simulink model "QD2_MissionCtrl_Dual_MPC"  (R2022b)
settings: Solver=ode2  StartTime=0.0  StopTime=inf  FixedStep=0.001  RelTol=1e-3  EnableMultiTasking=on
PreLoadFcn:
  | % Rutas: simulink_qdrone2 (qd2_cargar_config), lib (qd2_*.m) y la carpeta
  | % del modelo (QD2_Mission_Lib.slx de la misma versión de MATLAB).
  | qd2_d = fileparts(get_param(bdroot, 'FileName')); qd2_r = qd2_d;
  | while ~isempty(qd2_r) && ~exist(fullfile(qd2_r, 'qd2_cargar_config.m'), 'file')
  |     qd2_p = fileparts(qd2_r); if strcmp(qd2_p, qd2_r), qd2_r = ''; else, qd2_r = qd2_p; end
  | end
  | if ~isempty(qd2_r), addpath(fullfile(qd2_r, 'lib')); addpath(qd2_r); end
  | if exist(fullfile(qd2_d, 'QD2_Mission_Lib.slx'), 'file'), addpath(qd2_d); end
  | clear qd2_d qd2_r qd2_p
PostLoadFcn:
  | try, qd2_cargar_config(); catch qd2_e, warning(qd2_e.message); end
InitFcn:
  | qd2_cargar_config(bdroot);
undefined symbols (not defined in the file): _MissionCtrl, _MissionDual, datetime, Host, localhost, log_, m, qc_get_step_size, QD2CFG, QD2P, saved_data
libraries: quarc_library x43, QD2_Mission_Lib x12, simulink x11
(part 2 of 2)

== system QD2_MissionCtrl_Dual_MPC/MISSION CONTROL QDRONE POSITION CONTROL/Localization - Vicon ==
  note: Double-click on the Vicon block.
      |
      | Specify the Vicon Tracker server IP address and port number under Hostname field.
      |
      | Specify the object name corresponding to the vehicle to be tracked under the
      | List of segments field. The format for the segment is <ObjectName>.<ObjectName>
      | where <ObjectName> is the name given when defining the vehicle object in the
      | Vicon Tracker server softwre. Click the "+" button to add the name to the segment list
      | prior to clicking on the "OK" or "Apply" button.
      | Remove extra/unused entries from the list using the "-" button.
      |
      | Make sure the checkbox next to the Object name inside the Object tab in
      | Vicon Tracker software is selected/checked and Tracker is streaming (Live) tracking
      | data before running this model.
  Convention Correction (Vicon Frame to Research Studio Frame) : Subsystem  Commented=on
  For Each Subsystem (Convention Correction: Vicon Frame to Research Studio Frame) : Subsystem  TreatAsAtomicUnit=on
  Terminator{,1..4} (5 alike) : Terminator
  Vicon : quarc_library/Devices/Third-Party/Vicon/Vicon  hostname=localhost:801  segment_list=ObjectName1.ObjectName1\0\0  marker_list=\0  unlabeled_markers=[]  stream_mode=2  sample_time=qc_get_step_size  num_segments=1  num_markers=0  active=on
      settings: SourceProductName=QUARC Targets
  Data [7n] : Outport  VectorParamsAs1DForOutWhenUnconnected=off
  q [4n] : Outport  Port=2  VectorParamsAs1DForOutWhenUnconnected=off
  wires:
  Vicon/5 -> Terminator3/1
  Vicon/4 -> Terminator1/1
  Vicon/1 -> For Each Subsystem (Convention Correction: Vicon Frame to Research Studio Frame)/1(xyz_MF (m) [3n])
  Vicon/2 -> For Each Subsystem (Convention Correction: Vicon Frame to Research Studio Frame)/2(rot_MF (rad) [3n])
  Vicon/3 -> For Each Subsystem (Convention Correction: Vicon Frame to Research Studio Frame)/3(isTracking [n])
  For Each Subsystem (Convention Correction: Vicon Frame to Research Studio Frame)/5("data_RSF (m, rad, bool) [7n]") -> Data [7n]/1
  For Each Subsystem (Convention Correction: Vicon Frame to Research Studio Frame)/4(isTracking_RSF [n]) -> Terminator2/1
  For Each Subsystem (Convention Correction: Vicon Frame to Research Studio Frame)/3(rot_RSF (rad) [3n]) -> Terminator/1
  For Each Subsystem (Convention Correction: Vicon Frame to Research Studio Frame)/2(xyz_RSF (m) [3n]) -> Terminator4/1
  For Each Subsystem (Convention Correction: Vicon Frame to Research Studio Frame)/1(q_RSF [4n]) -> q [4n]/1

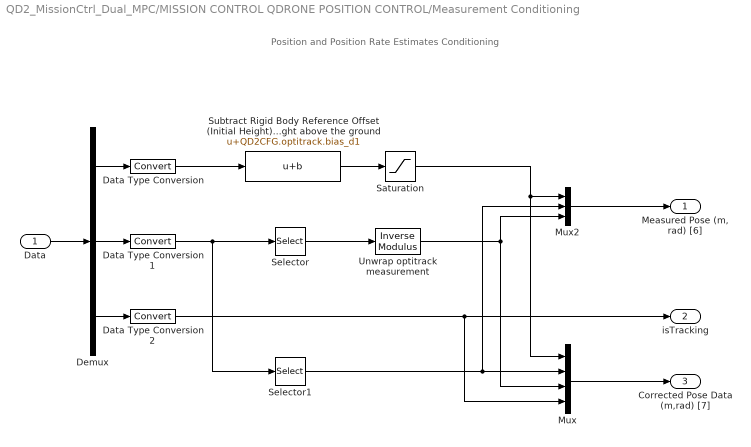
== system QD2_MissionCtrl_Dual_MPC/MISSION CONTROL QDRONE POSITION CONTROL/Measurement Conditioning ==
  note: Position and Position Rate Estimates Conditioning
  Data : Inport
  Data Type Conversion : DataTypeConversion  SaturateOnIntegerOverflow=off  RndMeth=Floor
  Data Type Conversion1 : DataTypeConversion  SaturateOnIntegerOverflow=off  RndMeth=Floor
  Data Type Conversion2 : DataTypeConversion  SaturateOnIntegerOverflow=off  RndMeth=Floor
  Demux : Demux  Outputs=[3 3 1]
  Mux : Mux
  Mux2 : Mux  Inputs=[3 2 1]
  Saturation : Saturate  UpperLimit=[2 2 5]  LowerLimit=[-2 -2 0]
  Selector : Selector  InputPortWidth=3  IndexOptions=Index vector (dialog)  Indices=[3]  OutputSizes=1
  Selector1 : Selector  InputPortWidth=3  IndexOptions=Index vector (dialog)  Indices=[1 2]  OutputSizes=1
  Subtract Rigid Body Reference Offset (Initial Height) to get height above the ground : Bias  Bias=QD2CFG.optitrack.bias_d1  SaturateOnIntegerOverflow=off
  Unwrap optitrack measurement : quarc_library/Discontinuities/Inverse Modulus  modulus=2*pi  output_derivative=off  output_revolutions=off  max_x=Inf  min_x=-Inf
  "Measured Pose (m, rad) [6]" : Outport  VectorParamsAs1DForOutWhenUnconnected=off
  isTracking : Outport  Port=2  VectorParamsAs1DForOutWhenUnconnected=off
  Corrected Pose Data (m,rad) [7] : Outport  Port=3  VectorParamsAs1DForOutWhenUnconnected=off
  wires:
  Demux/2 -> Data Type Conversion1/1
  Demux/1 -> Data Type Conversion/1
  Demux/3 -> Data Type Conversion2/1
  Mux2/1 -> "Measured Pose (m, rad) [6]"/1
  Data/1 -> Demux/1
  Data Type Conversion2/1 -> Mux/4, isTracking/1
  Subtract Rigid Body Reference Offset (Initial Height) to get height above the ground/1 -> Saturation/1
  Saturation/1 -> Mux2/1, Mux/1
  Data Type Conversion1/1 -> Selector1/1, Selector/1
  Selector/1 -> Unwrap optitrack measurement/1
  Data Type Conversion/1 -> Subtract Rigid Body Reference Offset (Initial Height) to get height above the ground/1
  Unwrap optitrack measurement/1 -> Mux2/3, Mux/3
  Mux/1 -> Corrected Pose Data (m,rad) [7]/1
  Selector1/1 -> Mux2/2, Mux/2

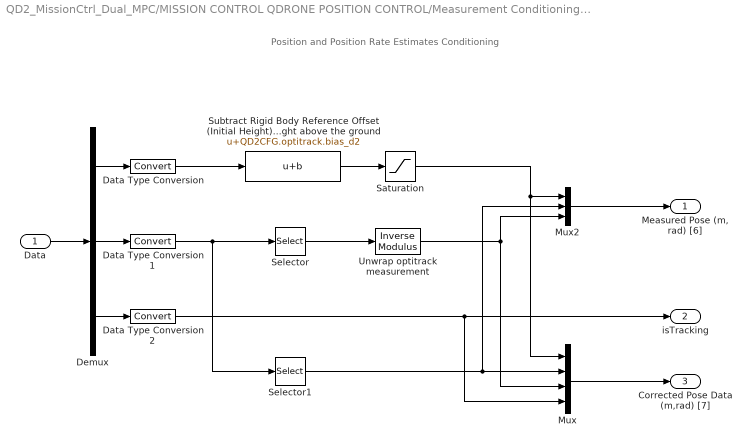
== system QD2_MissionCtrl_Dual_MPC/MISSION CONTROL QDRONE POSITION CONTROL/Measurement Conditioning QDrone 2 ==
  note: Position and Position Rate Estimates Conditioning
  Data : Inport
  Data Type Conversion : DataTypeConversion  SaturateOnIntegerOverflow=off  RndMeth=Floor
  Data Type Conversion1 : DataTypeConversion  SaturateOnIntegerOverflow=off  RndMeth=Floor
  Data Type Conversion2 : DataTypeConversion  SaturateOnIntegerOverflow=off  RndMeth=Floor
  Demux : Demux  Outputs=[3 3 1]
  Mux : Mux
  Mux2 : Mux  Inputs=[3 2 1]
  Saturation : Saturate  UpperLimit=[2 2 5]  LowerLimit=[-2 -2 0]
  Selector : Selector  InputPortWidth=3  IndexOptions=Index vector (dialog)  Indices=[3]  OutputSizes=1
  Selector1 : Selector  InputPortWidth=3  IndexOptions=Index vector (dialog)  Indices=[1 2]  OutputSizes=1
  Subtract Rigid Body Reference Offset (Initial Height) to get height above the ground : Bias  Bias=QD2CFG.optitrack.bias_d2  SaturateOnIntegerOverflow=off
  Unwrap optitrack measurement : quarc_library/Discontinuities/Inverse Modulus  modulus=2*pi  output_derivative=off  output_revolutions=off  max_x=Inf  min_x=-Inf
  "Measured Pose (m, rad) [6]" : Outport  VectorParamsAs1DForOutWhenUnconnected=off
  isTracking : Outport  Port=2  VectorParamsAs1DForOutWhenUnconnected=off
  Corrected Pose Data (m,rad) [7] : Outport  Port=3  VectorParamsAs1DForOutWhenUnconnected=off
  wires:
  Selector1/1 -> Mux/2, Mux2/2
  Mux/1 -> Corrected Pose Data (m,rad) [7]/1
  Unwrap optitrack measurement/1 -> Mux/3, Mux2/3
  Data Type Conversion/1 -> Subtract Rigid Body Reference Offset (Initial Height) to get height above the ground/1
  Selector/1 -> Unwrap optitrack measurement/1
  Data Type Conversion1/1 -> Selector/1, Selector1/1
  Saturation/1 -> Mux/1, Mux2/1
  Subtract Rigid Body Reference Offset (Initial Height) to get height above the ground/1 -> Saturation/1
  Data Type Conversion2/1 -> isTracking/1, Mux/4
  Data/1 -> Demux/1
  Mux2/1 -> "Measured Pose (m, rad) [6]"/1
  Demux/3 -> Data Type Conversion2/1
  Demux/1 -> Data Type Conversion/1
  Demux/2 -> Data Type Conversion1/1

== system QD2_MissionCtrl_Dual_MPC/MISSION CONTROL QDRONE POSITION CONTROL/Subsystem ==
  note: CORRECCIÓN (2 drones): el modelo de tierra ya no se detiene 3 s después de Land.
      | Stop Allowed (MISSION END CHECK) = los DOS drones en el suelo >= 3 s (o 60 s seguidos sin rastreo).
      | Después sigue el Delay original de 3 s y el Stop with Message.
  Joystick Signals (Boolean) : Inport
  "Communication Issue " : Inport  Port=2
  AND Stop Allowed : Logic  AllPortsSameDT=off  OutDataTypeStr=boolean
  Compare To Constant : simulink/Logic and Bit Operations/Compare To Constant  relop=>=  const=1  OutDataTypeStr=boolean
  Compare To Constant1 : simulink/Logic and Bit Operations/Compare To Constant  relop===  const=3  OutDataTypeStr=boolean
  Delay : Delay  DelayLength=3000
  Demux : Demux
  MATLAB Function : MATLAB Function  TreatAsAtomicUnit=on
  OR : Logic  Operator=OR  IconShape=distinctive  AllPortsSameDT=off  OutDataTypeStr=boolean
  Product : Product
  Stop with Message : quarc_library/Sinks/Error Handling/Stop with Message  message_type=Fixed error message  message_icon=Information  message=Mission plan ended, stopping mission control!
  Time : quarc_library/Sources/Time/Time  time_source=Wall clock  sample_time=qc_get_step_size
  Flight_State : Outport
  wires:
  Joystick Signals (Boolean)/1 -> Product/2
  Demux/1 -> MATLAB Function/1(Arm)
  Demux/2 -> MATLAB Function/2(Takeoff_Land_Flag)
  Demux/3 -> MATLAB Function/3(Emergency_Stop)
  Demux/4 -> MATLAB Function/4(Joystick_Issue)
  MATLAB Function/1(Flight_State) -> Flight_State/1, Compare To Constant1/1
  Product/1 -> Demux/1
  Time/1 -> Compare To Constant/1
  Compare To Constant/1 -> Product/1
  Delay/1 -> Stop with Message/1
  MATLAB Function/2(Stop_MS) -> OR/2
  Compare To Constant1/1 -> OR/1
  "Communication Issue "/1 -> MATLAB Function/5(Communication_Issue)
  OR/1 -> AND Stop Allowed/1
  [Stop_Allowed] -> AND Stop Allowed/2
  AND Stop Allowed/1 -> Delay/1

== system QD2_MissionCtrl_Dual_MPC/MISSION CONTROL QDRONE POSITION CONTROL/Subsystem QDrone 2 ==
  note: CORRECCIÓN (2 drones): el modelo de tierra ya no se detiene 3 s después de Land.
      | Stop Allowed (MISSION END CHECK) = los DOS drones en el suelo >= 3 s (o 60 s seguidos sin rastreo).
      | Después sigue el Delay original de 3 s y el Stop with Message.
  Joystick Signals (Boolean) : Inport
  "Communication Issue " : Inport  Port=2
  AND Stop Allowed : Logic  AllPortsSameDT=off  OutDataTypeStr=boolean
  Compare To Constant : simulink/Logic and Bit Operations/Compare To Constant  relop=>=  const=1  OutDataTypeStr=boolean
  Compare To Constant1 : simulink/Logic and Bit Operations/Compare To Constant  relop===  const=3  OutDataTypeStr=boolean
  Delay : Delay  DelayLength=3000
  Demux : Demux
  MATLAB Function : MATLAB Function  TreatAsAtomicUnit=on
  OR : Logic  Operator=OR  IconShape=distinctive  AllPortsSameDT=off  OutDataTypeStr=boolean
  Product : Product
  Stop with Message : quarc_library/Sinks/Error Handling/Stop with Message  message_type=Fixed error message  message_icon=Information  message=Mission plan ended, stopping mission control!
  Time : quarc_library/Sources/Time/Time  time_source=Wall clock  sample_time=qc_get_step_size
  Flight_State : Outport
  wires:
  AND Stop Allowed/1 -> Delay/1
  [Stop_Allowed] -> AND Stop Allowed/2
  OR/1 -> AND Stop Allowed/1
  "Communication Issue "/1 -> MATLAB Function/5(Communication_Issue)
  Compare To Constant1/1 -> OR/1
  MATLAB Function/2(Stop_MS) -> OR/2
  Delay/1 -> Stop with Message/1
  Compare To Constant/1 -> Product/1
  Time/1 -> Compare To Constant/1
  Product/1 -> Demux/1
  MATLAB Function/1(Flight_State) -> Compare To Constant1/1, Flight_State/1
  Demux/4 -> MATLAB Function/4(Joystick_Issue)
  Demux/3 -> MATLAB Function/3(Emergency_Stop)
  Demux/2 -> MATLAB Function/2(Takeoff_Land_Flag)
  Demux/1 -> MATLAB Function/1(Arm)
  Joystick Signals (Boolean)/1 -> Product/2

== system QD2_MissionCtrl_Dual_MPC/MISSION CONTROL QDRONE POSITION CONTROL/Triggered Subsystem ==
  note: This looks for the first falling edge of the communication issue before allowing a communication issue to be triggered,
      | because the mission server model starts first.
  Trigger : TriggerPort  TriggerType=falling  VariantControl=Variant
  Add : Sum
  Compare To Constant : simulink/Logic and Bit Operations/Compare To Constant  relop=>=  const=1  OutDataTypeStr=boolean
  Constant : Constant
  Memory : Memory  InheritSampleTime=on
  Communication Issue (0,1) : Outport  InitialOutput=0  VectorParamsAs1DForOutWhenUnconnected=off
  wires:
  Constant/1 -> Add/1
  Memory/1 -> Add/2
  Add/1 -> Compare To Constant/1, Memory/1
  Compare To Constant/1 -> Communication Issue (0,1)/1

== system QD2_MissionCtrl_Dual_MPC/MISSION CONTROL QDRONE POSITION CONTROL/Triggered Subsystem QDrone 2 ==
  note: This looks for the first falling edge of the communication issue before allowing a communication issue to be triggered,
      | because the mission server model starts first.
  Trigger : TriggerPort  TriggerType=falling  VariantControl=Variant
  Add : Sum
  Compare To Constant : simulink/Logic and Bit Operations/Compare To Constant  relop=>=  const=1  OutDataTypeStr=boolean
  Constant : Constant
  Memory : Memory  InheritSampleTime=on
  Communication Issue (0,1) : Outport  InitialOutput=0  VectorParamsAs1DForOutWhenUnconnected=off
  wires:
  Compare To Constant/1 -> Communication Issue (0,1)/1
  Add/1 -> Memory/1, Compare To Constant/1
  Memory/1 -> Add/2
  Constant/1 -> Add/1

== system QD2_MissionCtrl_Dual_MPC/MISSION CONTROL QDRONE POSITION CONTROL/Waypoint Trajectories ==
  note: Add waypoints as multiple rows of the RED matrix. The amount of time to wait at each waypoint is is defined as the coloumns of the GREEN row matrix.
      |
      | When Enable goes high, the vehicle will move to the first waypoint and wait there.
      | When Play/Pause goes high, the vehicle will spend time at the first waypoint (specified in the time vector) and then proceed to cycle through the remaining waypoints.
      | When Play/Pause goes low, the vehicle will pause at the current waypoint. If Play/Pause goes high again, it will resume by spending time at the corresponding waypoint
      | as specified in the time vector all over again.
      | When Enable goes low at any point, the vehicle will move back to the Default pose.
  Play/Pause : Inport
  "Default (m, rad) [4]" : Inport  Port=2
  Drone Pose (m,rad) [4] : Inport  Port=3
  Each row is a pose (Multiple rows are multiple poses) : Constant  Value=[0,0,1.0,0;-1.5,-1.5,1.0,0; 0,-1.5,1.0,0; 1.5,-1.5,1.0,0; -1.5,1.5,1.0,0;0 1.5 1.0 0; 1.5 1.5 1.0 0; 1.5 0.75 1.0 0; 0,0,1.0,0]  VectorParams1D=off
  Switch : Switch  Criteria=u2 > Threshold  SaturateOnIntegerOverflow=off  InputSameDT=off
  Waiting per location (s) (number of entries matches number of rows in position matrix above) : Constant  Value=5
  Waypoint_Generator : Subsystem
  Finished (0,1) : Outport
  "Trajectory (m, rad) [4]" : Outport  Port=2
  wires:
  Waypoint_Generator/2(Finished (0,1)) -> Finished (0,1)/1
  Switch/1 -> "Trajectory (m, rad) [4]"/1
  "Default (m, rad) [4]"/1 -> Switch/3
  Waypoint_Generator/1(Pose) -> Switch/1
  Play/Pause/1 -> Switch/2
  Each row is a pose (Multiple rows are multiple poses)/1 -> Waypoint_Generator/1(Pose Matrix)
  Drone Pose (m,rad) [4]/1 -> Waypoint_Generator/2(Drone Pose)
  Waiting per location (s) (number of entries matches number of rows in position matrix above)/1 -> Waypoint_Generator/3(Wait time)

== system QD2_MissionCtrl_Dual_MPC/MISSION CONTROL QDRONE POSITION CONTROL/Calculate Home Pose/Enabled Subsystem ==
  "Pose (m, rad ) [4] " : Inport
  Enable : EnablePort
  "Home Pose (m, rad ) [4]" : Outport  VectorParamsAs1DForOutWhenUnconnected=off
  wires:
  "Pose (m, rad ) [4] "/1 -> "Home Pose (m, rad ) [4]"/1

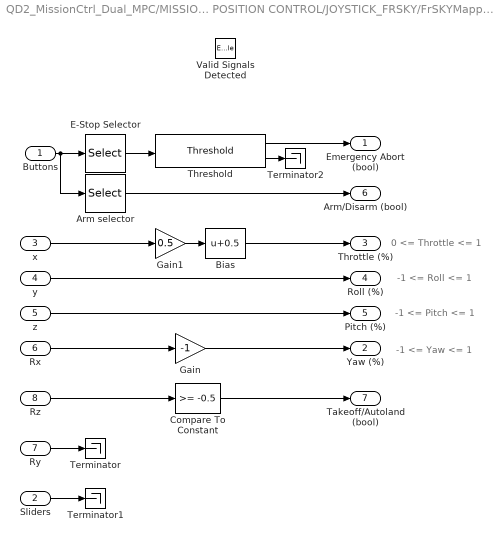
== system QD2_MissionCtrl_Dual_MPC/MISSION CONTROL QDRONE POSITION CONTROL/JOYSTICK_FRSKY/FrSKYMapping ==
  note: -1 <= Yaw <= 1
  note: 0 <= Throttle <= 1
  note: -1 <= Roll <= 1
  note: -1 <= Pitch <= 1
  Buttons : Inport
  Sliders : Inport  Port=2
  x : Inport  Port=3
  y : Inport  Port=4
  z : Inport  Port=5
  Rx : Inport  Port=6
  Ry : Inport  Port=7
  Rz : Inport  Port=8
  Valid Signals Detected : EnablePort
  Arm selector : Selector  InputPortWidth=32  IndexOptions=Index vector (dialog)  Indices=[2]  OutputSizes=1
  Bias : Bias  Bias=0.5  SaturateOnIntegerOverflow=off
  Compare To Constant : simulink/Logic and Bit Operations/Compare To Constant  relop=>=  const=-0.5  OutDataTypeStr=boolean
  E-Stop Selector : Selector  InputPortWidth=32  IndexOptions=Index vector (dialog)  Indices=[1]  OutputSizes=1
  Gain : Gain  Gain=-1
  Gain1 : Gain  Gain=0.5
  Terminator : Terminator
  Terminator1 : Terminator
  Terminator2 : Terminator
  Threshold : quarc_library/Discontinuities/Threshold  operator=>=  param_src=Specify via dialog  threshold=0.5  duration=0.2
      settings: SourceProductName=QUARC Targets
  Emergency Abort (bool) : Outport  VectorParamsAs1DForOutWhenUnconnected=off
  Yaw (%) : Outport  Port=2  VectorParamsAs1DForOutWhenUnconnected=off
  Throttle (%) : Outport  Port=3  VectorParamsAs1DForOutWhenUnconnected=off
  Roll (%) : Outport  Port=4  VectorParamsAs1DForOutWhenUnconnected=off
  Pitch (%) : Outport  Port=5  VectorParamsAs1DForOutWhenUnconnected=off
  "Arm/Disarm (bool) " : Outport  Port=6  VectorParamsAs1DForOutWhenUnconnected=off
  Takeoff/Autoland (bool) : Outport  Port=7  VectorParamsAs1DForOutWhenUnconnected=off
  wires:
  Buttons/1 -> Arm selector/1, E-Stop Selector/1
  Arm selector/1 -> "Arm/Disarm (bool) "/1
  x/1 -> Gain1/1
  y/1 -> Roll (%)/1
  z/1 -> Pitch (%)/1
  Rx/1 -> Gain/1
  Ry/1 -> Terminator/1
  Sliders/1 -> Terminator1/1
  E-Stop Selector/1 -> Threshold/1
  Rz/1 -> Compare To Constant/1
  Compare To Constant/1 -> Takeoff/Autoland (bool)/1
  Threshold/1 -> Emergency Abort (bool)/1
  Threshold/2 -> Terminator2/1
  Gain/1 -> Yaw (%)/1
  Gain1/1 -> Bias/1
  Bias/1 -> Throttle (%)/1

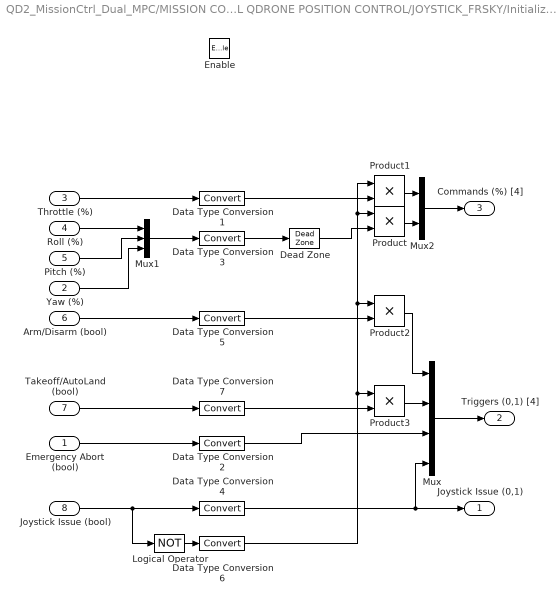
== system QD2_MissionCtrl_Dual_MPC/MISSION CONTROL QDRONE POSITION CONTROL/JOYSTICK_FRSKY/Initialization and Conditioning ==
  Emergency Abort (bool) : Inport
  Yaw (%) : Inport  Port=2
  Throttle (%) : Inport  Port=3
  Roll (%) : Inport  Port=4
  Pitch (%) : Inport  Port=5
  Arm/Disarm (bool) : Inport  Port=6
  Takeoff/AutoLand (bool) : Inport  Port=7
  Joystick Issue (bool) : Inport  Port=8
  Enable : EnablePort  StatesWhenEnabling=reset
  Data Type Conversion{1..7} (7 alike) : DataTypeConversion  SaturateOnIntegerOverflow=off  RndMeth=Floor
  Dead Zone : DeadZone  LowerValue=-0.01  UpperValue=0.01
  Logical Operator : Logic  Operator=NOT  AllPortsSameDT=off  OutDataTypeStr=boolean
  Mux : Mux
  Mux1 : Mux  Inputs=3
  Mux2 : Mux  Inputs=2
  Product{,1..3} (4 alike) : Product
  Joystick Issue (0,1) : Outport  InitialOutput=0  VectorParamsAs1DForOutWhenUnconnected=off
  Triggers (0,1) [4] : Outport  Port=2  InitialOutput=0  VectorParamsAs1DForOutWhenUnconnected=off
  Commands (%) [4] : Outport  Port=3  InitialOutput=0  VectorParamsAs1DForOutWhenUnconnected=off
  wires:
  Joystick Issue (bool)/1 -> Data Type Conversion4/1, Logical Operator/1
  Mux1/1 -> Data Type Conversion3/1
  Throttle (%)/1 -> Data Type Conversion1/1
  Roll (%)/1 -> Mux1/1
  Pitch (%)/1 -> Mux1/2
  Yaw (%)/1 -> Mux1/3
  Data Type Conversion4/1 -> Mux/4, Joystick Issue (0,1)/1
  Emergency Abort (bool)/1 -> Data Type Conversion2/1
  Data Type Conversion3/1 -> Dead Zone/1
  Arm/Disarm (bool)/1 -> Data Type Conversion5/1
  Mux/1 -> Triggers (0,1) [4]/1
  Data Type Conversion2/1 -> Mux/3
  Logical Operator/1 -> Data Type Conversion6/1
  Product/1 -> Mux2/2
  Product1/1 -> Mux2/1
  Data Type Conversion1/1 -> Product1/2
  Dead Zone/1 -> Product/2
  Data Type Conversion6/1 -> Product1/1, Product/1, Product2/1, Product3/1
  Product2/1 -> Mux/1
  Data Type Conversion5/1 -> Product2/2
  Takeoff/AutoLand (bool)/1 -> Data Type Conversion7/1
  Product3/1 -> Mux/2
  Data Type Conversion7/1 -> Product3/2
  Mux2/1 -> Commands (%) [4]/1

== system QD2_MissionCtrl_Dual_MPC/MISSION CONTROL QDRONE POSITION CONTROL/JOYSTICK_FRSKY/Pulse Check ==
  note: For this subsystem we will count the number of new pulses. The data can be considered enabled once the count of new signals has gone beyond 2. This will enable the Initializing and conditioning subsystem.
  new : Inport
  Compare : quarc_library/Logic Operations/Compare  operator=>=  output_data_type=boolean
      settings: SourceProductName=QUARC Targets
  Pulse Check : Constant
  "pulse count " : Subsystem  TreatAsAtomicUnit=on
  signal enable : Outport  InitialOutput=0  VectorParamsAs1DForOutWhenUnconnected=off
  wires:
  Compare/1 -> signal enable/1
  Pulse Check/1 -> Compare/2
  new/1 -> "pulse count "/Trigger
  "pulse count "/1(Number of Pulses) -> Compare/1

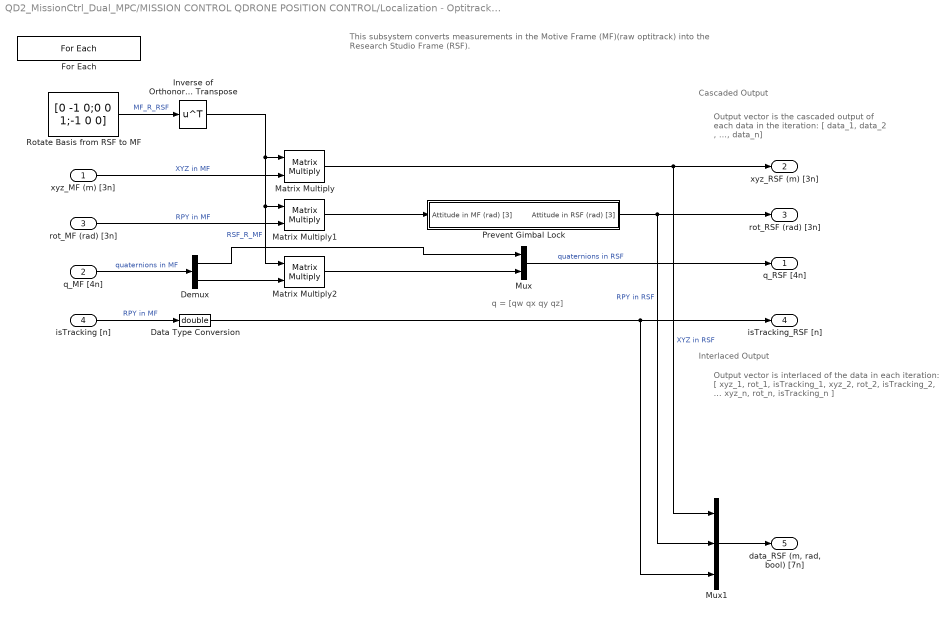
== system QD2_MissionCtrl_Dual_MPC/MISSION CONTROL QDRONE POSITION CONTROL/Localization - Optitrack/For Each Subsystem (Convention Correction: Motive Frame to Research Studio Frame) ==
  note: Output vector is interlaced of the data
      | in each iteration:
      |
      | [ xyz_1, rot_1, isTracking_1,
      |   xyz_2, rot_2, isTracking_2,
      |   ...
      |   xyz_n, rot_n, isTracking_n ]
  note: Interlaced Output
  note: Output vector is the cascaded output of
      | each data in the iteration:
      | [ data_1, data_2 , ..., data_n]
  note: Cascaded Output
  note: q = [qw qx qy qz]
  note: This subsystem converts measurements in the Motive Frame (MF)(raw optitrack) into the Research Studio Frame (RSF).
  xyz_MF (m) [3n] : Inport  Partition=on  PartitionDimension=1  PartitionWidth=3  PartitionOffset=0
  q_MF [4n] : Inport  Port=2  Partition=on  PartitionDimension=1  PartitionWidth=4  PartitionOffset=0
  rot_MF (rad) [3n] : Inport  Port=3  Partition=on  PartitionDimension=1  PartitionWidth=3  PartitionOffset=0
  isTracking [n] : Inport  Port=4  Partition=on  PartitionDimension=1  PartitionWidth=1  PartitionOffset=0
  Data Type Conversion : DataTypeConversion  OutDataTypeStr=double  SaturateOnIntegerOverflow=off  RndMeth=Floor
  Demux : Demux  Outputs=[1 3]
  For Each : ForEach  DisableCoverage=on
  Inverse of Orthonormal Matrix is its Transpose : Math  Operator=transpose
  Matrix Multiply : Product  Multiplication=Matrix(*)
  Matrix Multiply1 : Product  Multiplication=Matrix(*)
  Matrix Multiply2 : Product  Multiplication=Matrix(*)
  Mux : Mux  Inputs=2
  Mux1 : Mux  Inputs=3
  Prevent Gimbal Lock : Subsystem
  Rotate Basis from RSF to MF : Constant  Value=[0 -1 0;0 0 1;-1 0 0]
  q_RSF [4n] : Outport  ConcatenationDimension=1
  xyz_RSF (m) [3n] : Outport  Port=2  ConcatenationDimension=1
  rot_RSF (rad) [3n] : Outport  Port=3  ConcatenationDimension=1
  isTracking_RSF [n] : Outport  Port=4  ConcatenationDimension=1
  "data_RSF (m, rad, bool) [7n]" : Outport  Port=5  ConcatenationDimension=1
  wires:
  Mux/1 -> q_RSF [4n]/1  "quaternions in RSF"
  Demux/1 -> Mux/1
  Matrix Multiply2/1 -> Mux/2
  Demux/2 -> Matrix Multiply2/2
  q_MF [4n]/1 -> Demux/1  "quaternions in MF"
  Prevent Gimbal Lock/1(Attitude in RSF (rad) [3]) -> Mux1/2, rot_RSF (rad) [3n]/1  "RPY in RSF"
  Matrix Multiply1/1 -> Prevent Gimbal Lock/1(Attitude in MF (rad) [3])
  rot_MF (rad) [3n]/1 -> Matrix Multiply1/2  "RPY in MF"
  Matrix Multiply/1 -> Mux1/1, xyz_RSF (m) [3n]/1  "XYZ in RSF"
  Inverse of Orthonormal Matrix is its Transpose/1 -> Matrix Multiply/1, Matrix Multiply1/1, Matrix Multiply2/1  "RSF_R_MF"
  xyz_MF (m) [3n]/1 -> Matrix Multiply/2  "XYZ in MF"
  Rotate Basis from RSF to MF/1 -> Inverse of Orthonormal Matrix is its Transpose/1  "MF_R_RSF"
  isTracking [n]/1 -> Data Type Conversion/1  "RPY in MF"
  Mux1/1 -> "data_RSF (m, rad, bool) [7n]"/1
  Data Type Conversion/1 -> Mux1/3, isTracking_RSF [n]/1

== system QD2_MissionCtrl_Dual_MPC/MISSION CONTROL QDRONE POSITION CONTROL/Localization - Vicon/Convention Correction (Vicon Frame to Research Studio Frame) ==
  note: The VICON Global frame and the Research Studio Frame (RSF) are co-located and aligned.
      | The only mapping change is in the re-mapping of the Euler representation from
      | Relateive (Intrinsic) X-Y-Z to Relative Z-Y-X.
  xyz_global (m) [3] : Inport
  rot_global (rad) [3] : Inport  Port=2
  Demux : Demux  Outputs=3
  Euler Angles from Rotation Matrix (Relative ZYX) : quarc_library/Math Operations/Matrices/Euler Angles from Rotation Matrix  menu_order=Relative Z-Y-X
      settings: SourceProductName=QUARC Targets
  Euler Angles to Rotation Matrix (Relative XYZ) : quarc_library/Math Operations/Matrices/Euler Angles to Rotation Matrix  menu_order=Relative X-Y-Z
      settings: SourceProductName=QUARC Targets
  Inverse of Orthonormal Matrix : Math  Operator=transpose  SignedPower=on
  Mux : Mux  Inputs=3
  xyz_RSF (m) [3] : Outport  VectorParamsAs1DForOutWhenUnconnected=off
  rot_RSF (rad) [3] : Outport  Port=2  VectorParamsAs1DForOutWhenUnconnected=off
  R [3x3] : Outport  Port=3  VectorParamsAs1DForOutWhenUnconnected=off
  RT [3x3] : Outport  Port=4  VectorParamsAs1DForOutWhenUnconnected=off
  wires:
  Inverse of Orthonormal Matrix/1 -> RT [3x3]/1
  Euler Angles to Rotation Matrix (Relative XYZ)/1 -> Euler Angles from Rotation Matrix (Relative ZYX)/1, R [3x3]/1, Inverse of Orthonormal Matrix/1
  Euler Angles from Rotation Matrix (Relative ZYX)/2 -> Mux/2
  Euler Angles from Rotation Matrix (Relative ZYX)/3 -> Mux/1
  Mux/1 -> rot_RSF (rad) [3]/1
  Euler Angles from Rotation Matrix (Relative ZYX)/1 -> Mux/3
  xyz_global (m) [3]/1 -> xyz_RSF (m) [3]/1
  Demux/2 -> Euler Angles to Rotation Matrix (Relative XYZ)/2
  rot_global (rad) [3]/1 -> Demux/1
  Demux/1 -> Euler Angles to Rotation Matrix (Relative XYZ)/1
  Demux/3 -> Euler Angles to Rotation Matrix (Relative XYZ)/3

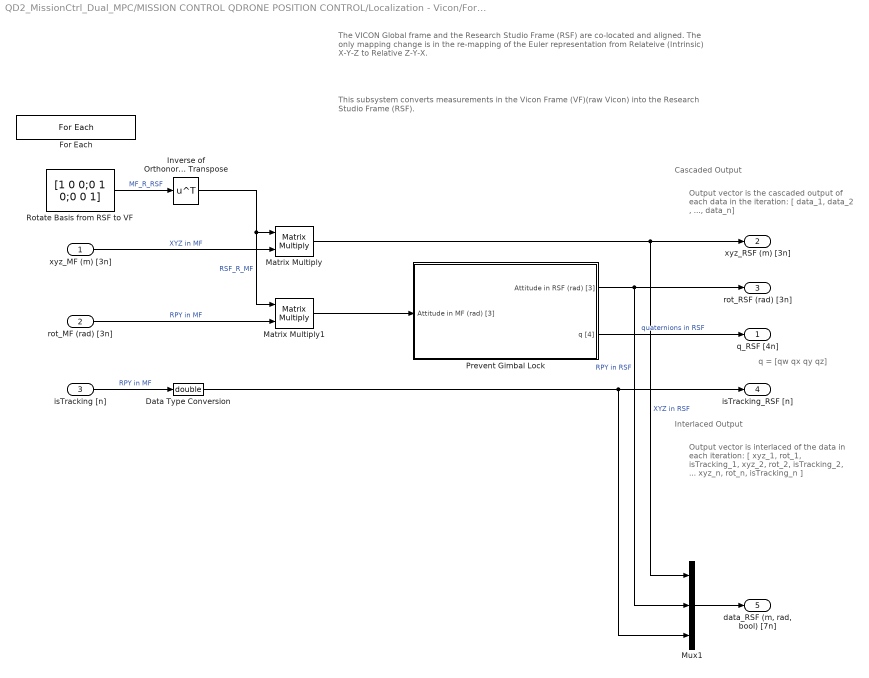
== system QD2_MissionCtrl_Dual_MPC/MISSION CONTROL QDRONE POSITION CONTROL/Localization - Vicon/For Each Subsystem (Convention Correction: Vicon Frame to Research Studio Frame) ==
  note: The VICON Global frame and the Research Studio Frame (RSF) are co-located and aligned.
      | The only mapping change is in the re-mapping of the Euler representation from
      | Relateive (Intrinsic) X-Y-Z to Relative Z-Y-X.
  note: Output vector is interlaced of the data
      | in each iteration:
      |
      | [ xyz_1, rot_1, isTracking_1,
      |   xyz_2, rot_2, isTracking_2,
      |   ...
      |   xyz_n, rot_n, isTracking_n ]
  note: Interlaced Output
  note: Output vector is the cascaded output of
      | each data in the iteration:
      | [ data_1, data_2 , ..., data_n]
  note: Cascaded Output
  note: q = [qw qx qy qz]
  note: This subsystem converts measurements in the Vicon Frame (VF)(raw Vicon) into the Research Studio Frame (RSF).
  xyz_MF (m) [3n] : Inport  Partition=on  PartitionDimension=1  PartitionWidth=3  PartitionOffset=0
  rot_MF (rad) [3n] : Inport  Port=2  Partition=on  PartitionDimension=1  PartitionWidth=3  PartitionOffset=0
  isTracking [n] : Inport  Port=3  Partition=on  PartitionDimension=1  PartitionWidth=3  PartitionOffset=0
  Data Type Conversion : DataTypeConversion  OutDataTypeStr=double  SaturateOnIntegerOverflow=off  RndMeth=Floor
  For Each : ForEach  DisableCoverage=on
  Inverse of Orthonormal Matrix is its Transpose : Math  Operator=transpose
  Matrix Multiply : Product  Multiplication=Matrix(*)
  Matrix Multiply1 : Product  Multiplication=Matrix(*)
  Mux1 : Mux  Inputs=3
  Prevent Gimbal Lock : Subsystem
  Rotate Basis from RSF to VF : Constant  Value=[1 0 0;0 1 0;0 0 1]
  q_RSF [4n] : Outport  ConcatenationDimension=1
  xyz_RSF (m) [3n] : Outport  Port=2  ConcatenationDimension=1
  rot_RSF (rad) [3n] : Outport  Port=3  ConcatenationDimension=1
  isTracking_RSF [n] : Outport  Port=4  ConcatenationDimension=1
  "data_RSF (m, rad, bool) [7n]" : Outport  Port=5  ConcatenationDimension=1
  wires:
  Prevent Gimbal Lock/2(q [4]) -> q_RSF [4n]/1  "quaternions in RSF"
  Prevent Gimbal Lock/1(Attitude in RSF (rad) [3]) -> Mux1/2, rot_RSF (rad) [3n]/1  "RPY in RSF"
  Matrix Multiply1/1 -> Prevent Gimbal Lock/1(Attitude in MF (rad) [3])
  rot_MF (rad) [3n]/1 -> Matrix Multiply1/2  "RPY in MF"
  Matrix Multiply/1 -> Mux1/1, xyz_RSF (m) [3n]/1  "XYZ in RSF"
  Inverse of Orthonormal Matrix is its Transpose/1 -> Matrix Multiply/1, Matrix Multiply1/1  "RSF_R_MF"
  xyz_MF (m) [3n]/1 -> Matrix Multiply/2  "XYZ in MF"
  Rotate Basis from RSF to VF/1 -> Inverse of Orthonormal Matrix is its Transpose/1  "MF_R_RSF"
  isTracking [n]/1 -> Data Type Conversion/1  "RPY in MF"
  Mux1/1 -> "data_RSF (m, rad, bool) [7n]"/1
  Data Type Conversion/1 -> Mux1/3, isTracking_RSF [n]/1

== system QD2_MissionCtrl_Dual_MPC/MISSION CONTROL QDRONE POSITION CONTROL/Waypoint Trajectories/Waypoint_Generator ==
  Pose Matrix : Inport
  Drone Pose : Inport  Port=2
  Wait time : Inport  Port=3
  Arrived : Subsystem
  MATLAB Function : MATLAB Function  TreatAsAtomicUnit=on
  Memory : Memory
  Timer : Subsystem
  Pose : Outport
  Finished (0,1) : Outport  Port=2
  wires:
  MATLAB Function/2(finished) -> Finished (0,1)/1
  Pose Matrix/1 -> MATLAB Function/1(waypoints_0)
  Drone Pose/1 -> Arrived/2(Drone Pose)
  Arrived/1(Arrived) -> Timer/2(arrived)
  MATLAB Function/1(waypoint) -> Arrived/1(Waypoint), Pose/1
  Timer/1(trigger) -> Memory/1
  Memory/1 -> MATLAB Function/2(trigger)
  Wait time/1 -> Timer/1(Wait time)

== system QD2_MissionCtrl_Dual_MPC/MISSION CONTROL QDRONE POSITION CONTROL/JOYSTICK_FRSKY/Pulse Check/pulse count  ==
  Trigger : TriggerPort  VariantControl=Variant
  Constant1 : Constant  Value=0
  Increment Stored Integer : simulink/Additional Math & Discrete/Additional Math: Increment - Decrement/Increment Stored Integer
  Sum : Sum  Inputs=|++
  Unit Delay : UnitDelay  SampleTime=-1  HasFrameUpgradeWarning=on
  Number of Pulses : Outport  VectorParamsAs1DForOutWhenUnconnected=off
  wires:
  Constant1/1 -> Sum/1
  Sum/1 -> Increment Stored Integer/1
  Unit Delay/1 -> Sum/2
  Increment Stored Integer/1 -> Unit Delay/1, Number of Pulses/1

== system QD2_MissionCtrl_Dual_MPC/MISSION CONTROL QDRONE POSITION CONTROL/Localization - Optitrack/For Each Subsystem (Convention Correction: Motive Frame to Research Studio Frame)/Prevent Gimbal Lock ==
  Attitude in MF (rad) [3] : Inport
  Demux : Demux  Outputs=3
  Euler Angles from Rotation Matrix (Relative ZYX) : quarc_library/Math Operations/Matrices/Euler Angles from Rotation Matrix  menu_order=Relative Z-Y-X
      settings: SourceProductName=QUARC Targets
  Euler Angles to Rotation Matrix (Relative YZX) : quarc_library/Math Operations/Matrices/Euler Angles to Rotation Matrix  menu_order=Relative Y-Z-X
      settings: SourceProductName=QUARC Targets
  Mux : Mux  Inputs=3
  Attitude in RSF (rad) [3] : Outport
  wires:
  Euler Angles to Rotation Matrix (Relative YZX)/1 -> Euler Angles from Rotation Matrix (Relative ZYX)/1
  Euler Angles from Rotation Matrix (Relative ZYX)/3 -> Mux/1
  Euler Angles from Rotation Matrix (Relative ZYX)/2 -> Mux/2
  Euler Angles from Rotation Matrix (Relative ZYX)/1 -> Mux/3
  Mux/1 -> Attitude in RSF (rad) [3]/1
  Demux/1 -> Euler Angles to Rotation Matrix (Relative YZX)/3
  Demux/3 -> Euler Angles to Rotation Matrix (Relative YZX)/2
  Demux/2 -> Euler Angles to Rotation Matrix (Relative YZX)/1
  Attitude in MF (rad) [3]/1 -> Demux/1

== system QD2_MissionCtrl_Dual_MPC/MISSION CONTROL QDRONE POSITION CONTROL/Localization - Vicon/For Each Subsystem (Convention Correction: Vicon Frame to Research Studio Frame)/Prevent Gimbal Lock ==
  Attitude in MF (rad) [3] : Inport
  Demux : Demux  Outputs=3
  Euler Angles from Rotation Matrix (Relative ZYX) : quarc_library/Math Operations/Matrices/Euler Angles from Rotation Matrix  menu_order=Relative Z-Y-X
      settings: SourceProductName=QUARC Targets
  Euler Angles to Rotation Matrix (Relative XYZ) : quarc_library/Math Operations/Matrices/Euler Angles to Rotation Matrix  menu_order=Relative X-Y-Z
      settings: SourceProductName=QUARC Targets
  Mux : Mux  Inputs=3
  Quaternion from Rotation Matrix : quarc_library/Math Operations/Quaternions/Quaternion from Rotation Matrix
      settings: SourceProductName=QUARC Targets
  Attitude in RSF (rad) [3] : Outport
  q [4] : Outport  Port=2
  wires:
  Euler Angles to Rotation Matrix (Relative XYZ)/1 -> Quaternion from Rotation Matrix/1, Euler Angles from Rotation Matrix (Relative ZYX)/1
  Euler Angles from Rotation Matrix (Relative ZYX)/3 -> Mux/1
  Euler Angles from Rotation Matrix (Relative ZYX)/2 -> Mux/2
  Euler Angles from Rotation Matrix (Relative ZYX)/1 -> Mux/3
  Mux/1 -> Attitude in RSF (rad) [3]/1
  Demux/1 -> Euler Angles to Rotation Matrix (Relative XYZ)/3
  Demux/3 -> Euler Angles to Rotation Matrix (Relative XYZ)/2
  Demux/2 -> Euler Angles to Rotation Matrix (Relative XYZ)/1
  Attitude in MF (rad) [3]/1 -> Demux/1
  Quaternion from Rotation Matrix/1 -> q [4]/1

== system QD2_MissionCtrl_Dual_MPC/MISSION CONTROL QDRONE POSITION CONTROL/Waypoint Trajectories/Waypoint_Generator/Arrived ==
  Waypoint : Inport
  Drone Pose : Inport  Port=2
  Constant : Constant  Value=0.1
  Dot Product : DotProduct  OutDataTypeStr=Inherit: Inherit via internal rule
  Memory : Memory
  Relational Operator1 : RelationalOperator  Operator=<=  OutDataTypeStr=boolean  InputSameDT=off
  Selector : Selector  InputPortWidth=4  IndexOptions=Index vector (dialog)  Indices=[1 2]  OutputSizes=1
  Selector1 : Selector  InputPortWidth=4  IndexOptions=Index vector (dialog)  Indices=[1 2]  OutputSizes=1
  Sqrt : Sqrt
  Sum : Sum  Inputs=|+-
  Arrived : Outport
  wires:
  Sum/1 -> Dot Product/2, Dot Product/1
  Selector1/1 -> Sum/1
  Selector/1 -> Sum/2
  Constant/1 -> Relational Operator1/2
  Relational Operator1/1 -> Memory/1
  Dot Product/1 -> Sqrt/1
  Memory/1 -> Arrived/1
  Sqrt/1 -> Relational Operator1/1
  Drone Pose/1 -> Selector/1
  Waypoint/1 -> Selector1/1

== system QD2_MissionCtrl_Dual_MPC/MISSION CONTROL QDRONE POSITION CONTROL/Waypoint Trajectories/Waypoint_Generator/Timer ==
  Wait time : Inport
  arrived : Inport  Port=2
  Cast To Double : DataTypeConversion  OutDataTypeStr=double  SaturateOnIntegerOverflow=off  RndMeth=Floor
  "Detect Rise Positive " : simulink/Logic and Bit Operations/Detect Rise Positive  vinit=0  OutDataTypeStr=boolean
  GreaterThan : RelationalOperator  Operator=<  OutDataTypeStr=boolean  RndMeth=Simplest  InputSameDT=off
  Integrator : Integrator  ExternalReset=falling
  Mux : Mux  Inputs=2
  Scope : Scope
  trigger : Outport
  wires:
  Integrator/1 -> GreaterThan/2
  Wait time/1 -> GreaterThan/1
  arrived/1 -> Cast To Double/1, Mux/2, Integrator/2
  GreaterThan/1 -> "Detect Rise Positive "/1
  Cast To Double/1 -> Integrator/1
  Mux/1 -> Scope/1
  "Detect Rise Positive "/1 -> trigger/1, Mux/1

== matlab function QD2_MissionCtrl_Dual_MPC/Communication QDrone 2/Detect Communication loss/MATLAB Function ==
  data: time input; stream_connection_loss output; state input; error input
function stream_connection_loss  = fcn(time, state, error)

stream_connection_loss = 0;
if time > 1
    if ~((state == 2)&&(error >= 0))
        % stream connection is not established correctly
        stream_connection_loss = 1;
    end
end

== matlab function QD2_MissionCtrl_Dual_MPC/MISSION CONTROL QDRONE POSITION CONTROL/Subsystem/MATLAB Function ==
  data: Arm input; Flight_State output; Takeoff_Land_Flag input; Emergency_Stop input; Joystick_Issue input; Stop_MS output; Communication_Issue input
function [Flight_State, Stop_MS]= Flight_Plan(Arm, ...
                            Takeoff_Land_Flag, ...
                            Emergency_Stop, ...
                            Joystick_Issue, ...
                            Communication_Issue)

persistent State

if isempty(State);
    State = 0;

end 
Stop_MS = 0;


switch State 

    case 0 % ============== QDrone Idle Sate ============== 
            
        if  Arm == 1 & Emergency_Stop == 0 && Joystick_Issue == 0
            State = 1;
        elseif Joystick_Issue == 1 || Emergency_Stop == 1 || Takeoff_Land_Flag == 1 || Communication_Issue == 1
            State = 9 ;
        end 

    case 1 % ============== QDrone Armed Sate ============== 
          if Emergency_Stop == 0 && Joystick_Issue == 0 
               if Arm == 0 
                     State = 0 ;
               elseif Arm == 1 && Takeoff_Land_Flag == 1 
                     State = 2 ;
                 end
              elseif Joystick_Issue == 1 || Communication_Issue == 1 || Emergency_Stop == 1
                State = 9 ;
        end 
          
    case 2 % ============== QDrone Takeoff Sate ============== 
          if Emergency_Stop == 0 && Joystick_Issue == 0 
               if Takeoff_Land_Flag == 0 
                State = 3 ;
              elseif Joystick_Issue == 1 || Arm == 0 || Communication_Issue == 1|| Emergency_Stop == 1
                State = 9 ;
               end 
          end 

    case 3 % ============== QDrone Land Sate ============== 
           if Joystick_Issue == 1 || Arm == 0 || Communication_Issue == 1
               State = 9 ;
           end

    case 9 % ============== MS Stop Sate ============== 
            Stop_MS = 1;
    
end 

Flight_State = State ;

== matlab function QD2_MissionCtrl_Dual_MPC/Communication QDrone 1/Detect Communication loss/MATLAB Function ==
  data: time input; stream_connection_loss output; state input; error input
function stream_connection_loss  = fcn(time, state, error)

stream_connection_loss = 0;
if time > 1
    if ~((state == 2)&&(error >= 0))
        % stream connection is not established correctly
        stream_connection_loss = 1;
    end
end

== matlab function QD2_MissionCtrl_Dual_MPC/MISSION CONTROL QDRONE POSITION CONTROL/Subsystem QDrone 2/MATLAB Function ==
  data: Arm input; Flight_State output; Takeoff_Land_Flag input; Emergency_Stop input; Joystick_Issue input; Stop_MS output; Communication_Issue input
function [Flight_State, Stop_MS]= Flight_Plan(Arm, ...
                            Takeoff_Land_Flag, ...
                            Emergency_Stop, ...
                            Joystick_Issue, ...
                            Communication_Issue)

persistent State

if isempty(State);
    State = 0;

end 
Stop_MS = 0;


switch State 

    case 0 % ============== QDrone Idle Sate ============== 
            
        if  Arm == 1 & Emergency_Stop == 0 && Joystick_Issue == 0
            State = 1;
        elseif Joystick_Issue == 1 || Emergency_Stop == 1 || Takeoff_Land_Flag == 1 || Communication_Issue == 1
            State = 9 ;
        end 

    case 1 % ============== QDrone Armed Sate ============== 
          if Emergency_Stop == 0 && Joystick_Issue == 0 
               if Arm == 0 
                     State = 0 ;
               elseif Arm == 1 && Takeoff_Land_Flag == 1 
                     State = 2 ;
                 end
              elseif Joystick_Issue == 1 || Communication_Issue == 1 || Emergency_Stop == 1
                State = 9 ;
        end 
          
    case 2 % ============== QDrone Takeoff Sate ============== 
          if Emergency_Stop == 0 && Joystick_Issue == 0 
               if Takeoff_Land_Flag == 0 
                State = 3 ;
              elseif Joystick_Issue == 1 || Arm == 0 || Communication_Issue == 1|| Emergency_Stop == 1
                State = 9 ;
               end 
          end 

    case 3 % ============== QDrone Land Sate ============== 
           if Joystick_Issue == 1 || Arm == 0 || Communication_Issue == 1
               State = 9 ;
           end

    case 9 % ============== MS Stop Sate ============== 
            Stop_MS = 1;
    
end 

Flight_State = State ;

== matlab function QD2_MissionCtrl_Dual_MPC/MISSION CONTROL QDRONE POSITION CONTROL/Waypoint Trajectories/Waypoint_Generator/MATLAB Function ==
  data: waypoints_0 input; waypoint output; trigger input; finished output
function [waypoint, finished]  = fcn(waypoints_0, trigger)
persistent idx status;
[m, ~] = size(waypoints_0);
finished = 0;
if isempty(idx)
    idx = 1;
    status = 0;
    
end

if trigger && idx < m && status == 0 
    idx = idx + 1;
end     
if  trigger && idx == m
    
    status = 1; 
    finished =1;
end 

waypoint = waypoints_0(idx, :);
